simulink model "gtm_design"  (R2021b)
settings: Solver=VariableStepAuto  StartTime=0.0  StopTime=10.0  MinStep=0.00999  RelTol=1e-3
StopFcn:
  | MWSout=grabmws(bdroot);
  | MWSout.lastrun=datestr(now);
values from neighbouring files (symbols this model uses):
  knots2fps = 1.68781    [setup.m]
  s = tf('s')    [setup.m]
undefined symbols (not defined in the file or in its folder): Aero, aftfuel, aftfuel_pos, AILL, AILLC, AILR, AILRC, alpha_deg, alt0, altitude_ft, Ax_g, Ay_g, Az_g, b, beta_deg, bias, BRAKEC, Cbar, cg_pos0, cg_shift_gear, ControlMode, DamageCase, DamageModels, DamageOnsetTime, deltc, Earth, ELLIB, ELLIBC, ELLOB, ELLOBC, ELRIB, ELRIBC, ELROB, ELROBC, engl_ang, engl_pos, engr_ang, engr_pos, etas0, etas1, etasc_feedthrough, FLAPLC, FLAPLIB, FLAPLOB, FLAPRC, FLAPRIB, FLAPROB, FlightMode, FuelUsed_Init, fwdfuel, fwdfuel_pos, GEAR, GEARC, Inertia0, Inertia_shift_gear, Ixx_model, Iyy_model, Izz_model, KTAS, LandingGear ... (+66)
libraries: simulink_extras x98, LPVBlockLibrary x54, simulink_need_slupdate x30, aerolibconvert2 x27, simulink x7, aerolibtransform2 x6, uavalgslib x4, UserContent_lib x2, robotcorelib x1, uavutilslib x1
(part 5 of 9)

== system gtm_design/Guidance/Heading Control/FlightState ==
  Feedback : Inport
  Bus Creator : BusCreator  Inputs=8
  Bus Selector : BusSelector  OutputSignals=AirData.KTAS
  Bus Selector1 : BusSelector  OutputSignals=MIDG.NAV_Vu_mps,MIDG.NAV_Vn_mps,MIDG.NAV_Ve_mps
  Bus Selector2 : BusSelector  OutputSignals=MIDG.NAV_Ve_mps,MIDG.NAV_Vn_mps
  Bus Selector3 : BusSelector  OutputSignals=MIDG.NAV_latitude_deg,MIDG.NAV_longitude_deg,MIDG.NAV_altitude_m
  Bus Selector4 : BusSelector  OutputSignals=MIDG.phi_deg,MAG3.p_deg
  Bus to Vector : BusToVector
  Bus to Vector1 : BusToVector
  Bus to Vector2 : BusToVector
  Constant1 : Constant  Value=[37.827926944;-75.494061666]
  Constant2 : Constant  Value=0
  Constant3 : Constant  Value=0
  Degrees to Radians{,1..3} (4 alike) : simulink_extras/Transformations/Degrees to Radians
  Demux1 : Demux  Outputs=3
      settings: DisplayOption=none
  Gain : Gain  Gain=-1
  LLA to Flat Earth : aerolibtransform2/LLA to Flat Earth  units=English  ptype=Earth (WGS84)  F=1/298.257223563  R=20925646.3255  refPosPort=on  LL0=[0 10]  psi=0
      settings: SourceProductBaseCode=AE
  Map 0_1 : Subsystem
  Mux : Mux  Inputs=2
  Mux2 : Mux  Inputs=2
  Trigonometric Function1 : Trigonometry  Operator=atan2
  Trigonometric Function3 : Trigonometry  Operator=atan2
  VecNorm : Subsystem
  Velocity Conversion : aerolibconvert2/Velocity Conversion  IU=kts  OU=m/s
  fpstoknots2 : Gain  Gain=180/pi
  FlightState : Outport
  wires:
  Degrees to Radians3/1 -> Bus Creator/8  "RollAngleRate"
  Degrees to Radians2/1 -> Bus Creator/7  "RollAngle"
  Degrees to Radians1/1 -> Bus Creator/6  "FlightPathAngle"
  Degrees to Radians/1 -> Bus Creator/5  "HeadingAngle"
  Bus Creator/1 -> FlightState/1
  Velocity Conversion/1 -> Bus Creator/4  "AirSpeed"
  Bus to Vector2/1 -> Degrees to Radians3/1  "RollAngleRate"
  Bus to Vector1/1 -> Degrees to Radians2/1  "RollAngle"
  Bus to Vector/1 -> Velocity Conversion/1  "KTAS"
  Bus Selector4/1 -> Bus to Vector1/1  "<phi_deg>"
  Bus Selector4/2 -> Bus to Vector2/1  "<p_deg>"
  fpstoknots2/1 -> Degrees to Radians1/1  "FlightPathAngle"
  Bus Selector/1 -> Bus to Vector/1  "<KTAS>"
  Demux1/1 -> Bus Creator/1  "North"
  Demux1/2 -> Bus Creator/2  "East"
  Gain/1 -> Bus Creator/3  "Height"
  Bus Selector1/1 -> Trigonometric Function1/1  "<NAV_Vu_mps>"
  Bus Selector1/2 -> Mux/1  "<NAV_Vn_mps>"
  Bus Selector1/3 -> Mux/2  "<NAV_Ve_mps>"
  Trigonometric Function1/1 -> fpstoknots2/1  "gamma"
  VecNorm/1(O) -> Trigonometric Function1/2
  Mux/1 -> VecNorm/1(I)
  Constant2/1 -> LLA to Flat Earth/5
  Demux1/3 -> Gain/1  "Down"
  Bus Selector3/3 -> LLA to Flat Earth/2  "<NAV_altitude_m>"
  Constant3/1 -> LLA to Flat Earth/3
  Bus Selector3/1 -> Mux2/1  "<NAV_latitude_deg>"
  Bus Selector3/2 -> Mux2/2  "<NAV_longitude_deg>"
  Constant1/1 -> LLA to Flat Earth/4
  LLA to Flat Earth/1 -> Demux1/1
  Mux2/1 -> LLA to Flat Earth/1
  Feedback/1 -> Bus Selector3/1, Bus Selector2/1, Bus Selector1/1, Bus Selector4/1, Bus Selector/1
  Bus Selector2/1 -> Trigonometric Function3/1  "<NAV_Ve_mps>"
  Map 0_1/1(O) -> Degrees to Radians/1  "HeadingAngle"
  Trigonometric Function3/1 -> Map 0_1/1(I)  "gndtrack"
  Bus Selector2/2 -> Trigonometric Function3/2  "<NAV_Vn_mps>"

== system gtm_design/Guidance/Heading Control/Windless ==
  Bus Creator : BusCreator  Inputs=4  OutDataTypeStr=Bus: FixedWingEnvironmentBus  NonVirtualBus=on
  Constant : Constant  Value=9.8066
  Constant1 : Constant  Value=0
  Constant2 : Constant  Value=0
  Constant3 : Constant  Value=0
  Environment : Outport  VectorParamsAs1DForOutWhenUnconnected=off
  wires:
  Constant/1 -> Bus Creator/4  "Gravity"
  Bus Creator/1 -> Environment/1
  Constant1/1 -> Bus Creator/1  "WindNorth"
  Constant3/1 -> Bus Creator/3  "WindDown"
  Constant2/1 -> Bus Creator/2  "WindEast"

== system gtm_design/Guidance/Orbit Following/Subsystem1 ==
  Feedback : Inport
  Bus Creator : BusCreator  Inputs=8
  Bus Selector : BusSelector  OutputSignals=AirData.KTAS
  Bus Selector1 : BusSelector  OutputSignals=MIDG.NAV_Vu_mps,MIDG.NAV_Vn_mps,MIDG.NAV_Ve_mps
  Bus Selector2 : BusSelector  OutputSignals=MIDG.NAV_Ve_mps,MIDG.NAV_Vn_mps
  Bus Selector3 : BusSelector  OutputSignals=MIDG.NAV_latitude_deg,MIDG.NAV_longitude_deg,MIDG.NAV_altitude_m
  Bus Selector4 : BusSelector  OutputSignals=MIDG.phi_deg,MAG3.p_deg
  Bus Selector6 : BusSelector  OutputSignals=North,East,Height,HeadingAngle  OutputAsBus=on
  Bus to Vector : BusToVector
  Bus to Vector1 : BusToVector
  Bus to Vector2 : BusToVector
  Constant1 : Constant  Value=[37.827926944;-75.494061666]
  Constant2 : Constant  Value=0
  Constant3 : Constant  Value=0
  Degrees to Radians{,1..3} (4 alike) : simulink_extras/Transformations/Degrees to Radians
  Demux1 : Demux  Outputs=3
      settings: DisplayOption=none
  Gain : Gain  Gain=-1
  LLA to Flat Earth : aerolibtransform2/LLA to Flat Earth  units=English  ptype=Earth (WGS84)  F=1/298.257223563  R=20925646.3255  refPosPort=on  LL0=[0 10]  psi=0
      settings: SourceProductBaseCode=AE
  Map 0_1 : Subsystem
  Mux : Mux  Inputs=2
  Mux2 : Mux  Inputs=2
  Trigonometric Function1 : Trigonometry  Operator=atan2
  Trigonometric Function3 : Trigonometry  Operator=atan2
  VecNorm : Subsystem
  Velocity Conversion : aerolibconvert2/Velocity Conversion  IU=kts  OU=m/s
  fpstoknots2 : Gain  Gain=180/pi
  Out2 : Outport
  Out1 : Outport  Port=2
  wires:
  Bus Selector2/2 -> Trigonometric Function3/2  "<NAV_Vn_mps>"
  Trigonometric Function3/1 -> Map 0_1/1(I)  "gndtrack"
  Map 0_1/1(O) -> Degrees to Radians/1  "HeadingAngle"
  Bus Selector2/1 -> Trigonometric Function3/1  "<NAV_Ve_mps>"
  Feedback/1 -> Bus Selector/1, Bus Selector4/1, Bus Selector1/1, Bus Selector2/1, Bus Selector3/1
  Mux2/1 -> LLA to Flat Earth/1
  LLA to Flat Earth/1 -> Demux1/1
  Constant1/1 -> LLA to Flat Earth/4
  Bus Selector3/2 -> Mux2/2  "<NAV_longitude_deg>"
  Bus Selector3/1 -> Mux2/1  "<NAV_latitude_deg>"
  Constant3/1 -> LLA to Flat Earth/3
  Bus Selector3/3 -> LLA to Flat Earth/2  "<NAV_altitude_m>"
  Demux1/3 -> Gain/1  "Down"
  Constant2/1 -> LLA to Flat Earth/5
  Mux/1 -> VecNorm/1(I)
  VecNorm/1(O) -> Trigonometric Function1/2
  Trigonometric Function1/1 -> fpstoknots2/1  "gamma"
  Bus Selector1/3 -> Mux/2  "<NAV_Ve_mps>"
  Bus Selector1/2 -> Mux/1  "<NAV_Vn_mps>"
  Bus Selector1/1 -> Trigonometric Function1/1  "<NAV_Vu_mps>"
  Gain/1 -> Bus Creator/3  "Height"
  Demux1/2 -> Bus Creator/2  "East"
  Demux1/1 -> Bus Creator/1  "North"
  Bus Selector/1 -> Bus to Vector/1  "<KTAS>"
  fpstoknots2/1 -> Degrees to Radians1/1  "FlightPathAngle"
  Bus Selector4/2 -> Bus to Vector2/1  "<p_deg>"
  Bus Selector4/1 -> Bus to Vector1/1  "<phi_deg>"
  Bus to Vector/1 -> Velocity Conversion/1  "KTAS"
  Bus to Vector1/1 -> Degrees to Radians2/1  "RollAngle"
  Bus to Vector2/1 -> Degrees to Radians3/1  "RollAngleRate"
  Velocity Conversion/1 -> Bus Creator/4  "AirSpeed"
  Bus Selector6/1 -> Out1/1
  Bus Creator/1 -> Bus Selector6/1, Out2/1
  Degrees to Radians/1 -> Bus Creator/5  "HeadingAngle"
  Degrees to Radians1/1 -> Bus Creator/6  "FlightPathAngle"
  Degrees to Radians2/1 -> Bus Creator/7  "RollAngle"
  Degrees to Radians3/1 -> Bus Creator/8  "RollAngleRate"

== system gtm_design/Guidance/Orbit Following/Windless ==
  Bus Creator : BusCreator  Inputs=4  OutDataTypeStr=Bus: FixedWingEnvironmentBus  NonVirtualBus=on
  Constant : Constant  Value=9.8066
  Constant1 : Constant  Value=0
  Constant2 : Constant  Value=0
  Constant3 : Constant  Value=0
  Environment : Outport  VectorParamsAs1DForOutWhenUnconnected=off
  wires:
  Constant2/1 -> Bus Creator/2  "WindEast"
  Constant3/1 -> Bus Creator/3  "WindDown"
  Constant1/1 -> Bus Creator/1  "WindNorth"
  Bus Creator/1 -> Environment/1
  Constant/1 -> Bus Creator/4  "Gravity"

== system gtm_design/Guidance/Waypoint Following/Subsystem1 ==
  Feedback : Inport
  Bus Creator : BusCreator  Inputs=8
  Bus Selector : BusSelector  OutputSignals=AirData.KTAS
  Bus Selector1 : BusSelector  OutputSignals=MIDG.NAV_Vu_mps,MIDG.NAV_Vn_mps,MIDG.NAV_Ve_mps
  Bus Selector2 : BusSelector  OutputSignals=MIDG.NAV_Ve_mps,MIDG.NAV_Vn_mps
  Bus Selector3 : BusSelector  OutputSignals=MIDG.NAV_latitude_deg,MIDG.NAV_longitude_deg,MIDG.NAV_altitude_m
  Bus Selector4 : BusSelector  OutputSignals=MIDG.phi_deg,MAG3.p_deg
  Bus Selector6 : BusSelector  OutputSignals=North,East,Height,HeadingAngle  OutputAsBus=on
  Bus to Vector : BusToVector
  Bus to Vector1 : BusToVector
  Bus to Vector2 : BusToVector
  Constant1 : Constant  Value=[37.827926944;-75.494061666]
  Constant2 : Constant  Value=0
  Constant3 : Constant  Value=0
  Degrees to Radians{,1..3} (4 alike) : simulink_extras/Transformations/Degrees to Radians
  Demux1 : Demux  Outputs=3
      settings: DisplayOption=none
  Gain : Gain  Gain=-1
  LLA to Flat Earth : aerolibtransform2/LLA to Flat Earth  units=English  ptype=Earth (WGS84)  F=1/298.257223563  R=20925646.3255  refPosPort=on  LL0=[0 10]  psi=0
      settings: SourceProductBaseCode=AE
  Map 0_1 : Subsystem
  Mux : Mux  Inputs=2
  Mux2 : Mux  Inputs=2
  Trigonometric Function1 : Trigonometry  Operator=atan2
  Trigonometric Function3 : Trigonometry  Operator=atan2
  VecNorm : Subsystem
  Velocity Conversion : aerolibconvert2/Velocity Conversion  IU=kts  OU=m/s
  fpstoknots2 : Gain  Gain=180/pi
  Out2 : Outport
  Out1 : Outport  Port=2
  wires:
  Degrees to Radians3/1 -> Bus Creator/8  "RollAngleRate"
  Degrees to Radians2/1 -> Bus Creator/7  "RollAngle"
  Degrees to Radians1/1 -> Bus Creator/6  "FlightPathAngle"
  Degrees to Radians/1 -> Bus Creator/5  "HeadingAngle"
  Bus Creator/1 -> Out2/1, Bus Selector6/1
  Bus Selector6/1 -> Out1/1
  Velocity Conversion/1 -> Bus Creator/4  "AirSpeed"
  Bus to Vector2/1 -> Degrees to Radians3/1  "RollAngleRate"
  Bus to Vector1/1 -> Degrees to Radians2/1  "RollAngle"
  Bus to Vector/1 -> Velocity Conversion/1  "KTAS"
  Bus Selector4/1 -> Bus to Vector1/1  "<phi_deg>"
  Bus Selector4/2 -> Bus to Vector2/1  "<p_deg>"
  fpstoknots2/1 -> Degrees to Radians1/1  "FlightPathAngle"
  Bus Selector/1 -> Bus to Vector/1  "<KTAS>"
  Demux1/1 -> Bus Creator/1  "North"
  Demux1/2 -> Bus Creator/2  "East"
  Gain/1 -> Bus Creator/3  "Height"
  Bus Selector1/1 -> Trigonometric Function1/1  "<NAV_Vu_mps>"
  Bus Selector1/2 -> Mux/1  "<NAV_Vn_mps>"
  Bus Selector1/3 -> Mux/2  "<NAV_Ve_mps>"
  Trigonometric Function1/1 -> fpstoknots2/1  "gamma"
  VecNorm/1(O) -> Trigonometric Function1/2
  Mux/1 -> VecNorm/1(I)
  Constant2/1 -> LLA to Flat Earth/5
  Demux1/3 -> Gain/1  "Down"
  Bus Selector3/3 -> LLA to Flat Earth/2  "<NAV_altitude_m>"
  Constant3/1 -> LLA to Flat Earth/3
  Bus Selector3/1 -> Mux2/1  "<NAV_latitude_deg>"
  Bus Selector3/2 -> Mux2/2  "<NAV_longitude_deg>"
  Constant1/1 -> LLA to Flat Earth/4
  LLA to Flat Earth/1 -> Demux1/1
  Mux2/1 -> LLA to Flat Earth/1
  Feedback/1 -> Bus Selector3/1, Bus Selector2/1, Bus Selector1/1, Bus Selector4/1, Bus Selector/1
  Bus Selector2/1 -> Trigonometric Function3/1  "<NAV_Ve_mps>"
  Map 0_1/1(O) -> Degrees to Radians/1  "HeadingAngle"
  Trigonometric Function3/1 -> Map 0_1/1(I)  "gndtrack"
  Bus Selector2/2 -> Trigonometric Function3/2  "<NAV_Vn_mps>"

== system gtm_design/Guidance/Waypoint Following/Windless ==
  Bus Creator : BusCreator  Inputs=4  OutDataTypeStr=Bus: FixedWingEnvironmentBus  NonVirtualBus=on
  Constant : Constant  Value=9.8066
  Constant1 : Constant  Value=0
  Constant2 : Constant  Value=0
  Constant3 : Constant  Value=0
  Environment : Outport  VectorParamsAs1DForOutWhenUnconnected=off
  wires:
  Constant/1 -> Bus Creator/4  "Gravity"
  Bus Creator/1 -> Environment/1
  Constant1/1 -> Bus Creator/1  "WindNorth"
  Constant3/1 -> Bus Creator/3  "WindDown"
  Constant2/1 -> Bus Creator/2  "WindEast"

== system gtm_design/Control/Controller/Control Algorithm/Hinf Autopilot ==
  cmd : Inport
  feedback : Inport  Port=2
  Action Port : ActionPort  ActionPortLabel=case [ 3 ]:
  Bus Selector : BusSelector  OutputSignals=tas_c_knot,alt_c_ft,bet_c_deg,phi_c_deg  OutputAsBus=on
  Lateral-Directional Controller : Subsystem
  Longitudinal Controller : Subsystem
  Mux : Mux  Inputs=5
  CONTROLC : Outport  PortDimensions=[5 1]  InitialOutput=zeros(5,1)
  wires:
  Mux/1 -> CONTROLC/1
  Lateral-Directional Controller/1(AILC) -> Mux/3
  Lateral-Directional Controller/2(RUDC) -> Mux/4
  Longitudinal Controller/1(THROTC) -> Mux/1
  Longitudinal Controller/2(ELLC) -> Mux/2
  Lateral-Directional Controller/3(SPANAC) -> Mux/5
  feedback/1 -> Lateral-Directional Controller/2(feedback), Longitudinal Controller/2(feedback)
  Bus Selector/1 -> Lateral-Directional Controller/1(cmd_autopilot_lat), Longitudinal Controller/1(cmd_autopilot_lon)
  cmd/1 -> Bus Selector/1

== system gtm_design/Control/Controller/Control Algorithm/Hinf CAS ==
  cmd : Inport
  feedback : Inport  Port=2
  Action Port : ActionPort  ActionPortLabel=case [ 1 ]:
  Bus Selector : BusSelector  OutputSignals=an_c_g,bet_c_deg,p_c_deg  OutputAsBus=on
  Lateral-Directional Controller : Subsystem
  Longitudinal Controller : Subsystem
  Mux : Mux  Inputs=5
  CONTROLC : Outport  PortDimensions=[5 1]  InitialOutput=zeros(5,1)
  wires:
  cmd/1 -> Bus Selector/1
  Bus Selector/1 -> Longitudinal Controller/1(cmd_cas_lon), Lateral-Directional Controller/1(cmd_cas_lat)
  feedback/1 -> Longitudinal Controller/2(feedback), Lateral-Directional Controller/2(feedback)
  Lateral-Directional Controller/3(SPANAC) -> Mux/5
  Longitudinal Controller/2(ELLC) -> Mux/2
  Longitudinal Controller/1(THROTC) -> Mux/1
  Lateral-Directional Controller/2(RUDC) -> Mux/4
  Lateral-Directional Controller/1(AILC) -> Mux/3
  Mux/1 -> CONTROLC/1

== system gtm_design/Control/Controller/Control Algorithm/LPV Autopilot ==
  cmd : Inport
  feedback : Inport  Port=2
  Action Port : ActionPort  ActionPortLabel=case [ 4 ]:
  Bus Selector : BusSelector  OutputSignals=tas_c_knot,alt_c_ft,bet_c_deg,phi_c_deg  OutputAsBus=on
  Lateral-Directional Controller : Subsystem
  Longitudinal Controller : Subsystem
  Mux : Mux  Inputs=5
  CONTROLC : Outport  PortDimensions=[5 1]  InitialOutput=zeros(5,1)
  wires:
  Bus Selector/1 -> Longitudinal Controller/1(cmd_autopilot_lon), Lateral-Directional Controller/1(cmd_autopilot_lat)
  feedback/1 -> Longitudinal Controller/2(feedback), Lateral-Directional Controller/2(feedback)
  Lateral-Directional Controller/3(SPANAC) -> Mux/5
  Longitudinal Controller/2(ELLC) -> Mux/2
  Longitudinal Controller/1(THROTC) -> Mux/1
  Lateral-Directional Controller/2(RUDC) -> Mux/4
  Lateral-Directional Controller/1(AILC) -> Mux/3
  Mux/1 -> CONTROLC/1
  cmd/1 -> Bus Selector/1

== system gtm_design/Control/Controller/Control Algorithm/LPV CAS ==
  cmd : Inport
  feedback : Inport  Port=2
  Action Port : ActionPort  ActionPortLabel=case [ 2 ]:
  Bus Selector : BusSelector  OutputSignals=an_c_g,bet_c_deg,p_c_deg  OutputAsBus=on
  Lateral-Directional Controller : Subsystem
  Longitudinal Controller : Subsystem
  Mux : Mux  Inputs=5
  CONTROLC : Outport  PortDimensions=[5 1]  InitialOutput=zeros(5,1)
  wires:
  Mux/1 -> CONTROLC/1
  Lateral-Directional Controller/1(AILC) -> Mux/3
  Lateral-Directional Controller/2(RUDC) -> Mux/4
  Longitudinal Controller/1(THROTC) -> Mux/1
  Longitudinal Controller/2(ELLC) -> Mux/2
  Lateral-Directional Controller/3(SPANAC) -> Mux/5
  feedback/1 -> Lateral-Directional Controller/2(feedback), Longitudinal Controller/2(feedback)
  Bus Selector/1 -> Lateral-Directional Controller/1(cmd_cas_lat), Longitudinal Controller/1(cmd_cas_lon)
  cmd/1 -> Bus Selector/1

== system gtm_design/Control/Controller/Control Algorithm/No Control ==
  Action Port : ActionPort  ActionPortLabel=default:
  Elevator : Constant  Value=bias.elevator
  Flaps1 : Constant  Value=bias.rudder
  Flaps2 : Constant  Value=bias.aileron
  Flaps3 : Constant  Value=0
  Mux : Mux  Inputs=5
  Throttle : Constant  Value=bias.throttle
  CONTROLC : Outport  PortDimensions=[5 1]  InitialOutput=zeros(5,1)
  wires:
  Throttle/1 -> Mux/1
  Elevator/1 -> Mux/2
  Flaps2/1 -> Mux/3
  Flaps1/1 -> Mux/4
  Flaps3/1 -> Mux/5
  Mux/1 -> CONTROLC/1

== system gtm_design/GTM_T2/A//C parameters/Inertia//Mass//CG Shift/DamageEffects ==
  In : Inport
  Gain1 : Constant  Value=dInertiaDamage
  Squeeze2 : Squeeze
  Value(ndx,:) : Selector  NumberOfDimensions=2  IndexMode=Zero-based  InputPortWidth=3  IndexOptions=Index vector (port),Select all  Indices=[1 3],1  OutputSizes=1,1
  dInertia : Outport
  wires:
  Squeeze2/1 -> dInertia/1
  Value(ndx,:)/1 -> Squeeze2/1
  Gain1/1 -> Value(ndx,:)/1
  In/1 -> Value(ndx,:)/2

== system gtm_design/GTM_T2/A//C parameters/Inertia//Mass//CG Shift/FuelBurnEffects ==
  In : Inport
  Mux : Mux
  Polyval : Subsystem  mask{p=Ixx_model}
      mask prompts: p "Polynomial"
      mask help:
      | Embedded MATLAB version of the polyval block.
      | Input polynomial coefficients as a vector in descending order.
      mask Display:
      | disp('y = P(u)\n')
      | disp(['\nO(P) = ' num2str(length(p)-1)])
  Polyval1 : Subsystem  mask{p=Iyy_model}
      mask prompts: p "Polynomial"
      mask help:
      | Embedded MATLAB version of the polyval block.
      | Input polynomial coefficients as a vector in descending order.
      mask Display:
      | disp('y = P(u)\n')
      | disp(['\nO(P) = ' num2str(length(p)-1)])
  Polyval2 : Subsystem  mask{p=Izz_model}
      mask prompts: p "Polynomial"
      mask help:
      | Embedded MATLAB version of the polyval block.
      | Input polynomial coefficients as a vector in descending order.
      mask Display:
      | disp('y = P(u)\n')
      | disp(['\nO(P) = ' num2str(length(p)-1)])
  xCG6 : Constant  Value=zeros(1,3)
  dInertia : Outport
  wires:
  Mux/1 -> dInertia/1
  Polyval2/1(Out1) -> Mux/3
  Polyval1/1(Out1) -> Mux/2
  Polyval/1(Out1) -> Mux/1
  xCG6/1 -> Mux/4
  In/1 -> Polyval2/1(In1), Polyval1/1(In1), Polyval/1(In1)

== system gtm_design/GTM_T2/A//C parameters/Inertia//Mass//CG Shift/MorphingEffects ==
  morphing : Inport
  MorphingEffectsInertia : MATLAB Function  TreatAsAtomicUnit=on
  dInertia : Outport
  dCG : Outport  Port=2
  wires:
  morphing/1 -> MorphingEffectsInertia/1(eta)
  MorphingEffectsInertia/1(dinertia) -> dInertia/1
  MorphingEffectsInertia/2(dCG) -> dCG/1

== system gtm_design/GTM_T2/A//C parameters/Inertia//Mass//CG Shift/cg//weight ==
  DamageCase : Inport
  Gain1 : Constant  Value=dMassDamage
  Gain2 : Constant  Value=dCGDamage
  Squeeze1 : Squeeze
  Squeeze2 : Squeeze
  Value(ndx,:) : Selector  IndexMode=Zero-based  IndexOptions=Index vector (port)  Indices=[1 3]  OutputSizes=1
  Value(ndx,:)1 : Selector  NumberOfDimensions=2  IndexMode=Zero-based  InputPortWidth=3  IndexOptions=Index vector (port),Select all  Indices=[1 3],1  OutputSizes=1,1
  dCG : Outport
  dweight : Outport  Port=2
  wires:
  Squeeze2/1 -> dweight/1
  Squeeze1/1 -> dCG/1
  Value(ndx,:)/1 -> Squeeze2/1
  Gain1/1 -> Value(ndx,:)/1
  DamageCase/1 -> Value(ndx,:)1/2, Value(ndx,:)/2
  Value(ndx,:)1/1 -> Squeeze1/1
  Gain2/1 -> Value(ndx,:)1/1

== system gtm_design/GTM_T2/Actuators/Acutator Dynamics/ElevatorLIBServo ==
  In : Inport
  Constant : Constant  Value=Bias
  Gain : Gain  Gain=2*pi*freq  SaturateOnIntegerOverflow=on  OutDataTypeStr=Inherit: Same as input  ParamDataTypeStr=Inherit: Same as input
  Integrator : Integrator  InitialConditionSource=external  LimitOutput=on  UpperSaturationLimit=POS_hi  LowerSaturationLimit=POS_lo  IgnoreLimit=on
  Rate Limiter : Saturate  UpperLimit=RL  LowerLimit=-RL
  Sum : Sum  Inputs=-+|  InputSameDT=on  SaturateOnIntegerOverflow=on  OutDataTypeStr=Inherit: Same as first input
  Sum1 : Sum  Inputs=++|  InputSameDT=on  SaturateOnIntegerOverflow=on  OutDataTypeStr=Inherit: Same as first input
  Out : Outport  PortDimensions=1
  wires:
  Constant/1 -> Sum1/1
  Sum1/1 -> Integrator/2, Sum/2
  In/1 -> Sum1/2
  Rate Limiter/1 -> Integrator/1  "Ydot_lim"
  Integrator/1 -> Out/1, Sum/1  "Y"
  Sum/1 -> Gain/1  "Error"
  Gain/1 -> Rate Limiter/1  "Ydot"

== system gtm_design/GTM_T2/Actuators/Acutator Dynamics/ElevatorLOBServo ==
  In : Inport
  Constant : Constant  Value=Bias
  Gain : Gain  Gain=2*pi*freq  SaturateOnIntegerOverflow=on  OutDataTypeStr=Inherit: Same as input  ParamDataTypeStr=Inherit: Same as input
  Integrator : Integrator  InitialConditionSource=external  LimitOutput=on  UpperSaturationLimit=POS_hi  LowerSaturationLimit=POS_lo  IgnoreLimit=on
  Rate Limiter : Saturate  UpperLimit=RL  LowerLimit=-RL
  Sum : Sum  Inputs=-+|  InputSameDT=on  SaturateOnIntegerOverflow=on  OutDataTypeStr=Inherit: Same as first input
  Sum1 : Sum  Inputs=++|  InputSameDT=on  SaturateOnIntegerOverflow=on  OutDataTypeStr=Inherit: Same as first input
  Out : Outport  PortDimensions=1
  wires:
  Constant/1 -> Sum1/1
  Sum1/1 -> Integrator/2, Sum/2
  In/1 -> Sum1/2
  Rate Limiter/1 -> Integrator/1  "Ydot_lim"
  Integrator/1 -> Out/1, Sum/1  "Y"
  Sum/1 -> Gain/1  "Error"
  Gain/1 -> Rate Limiter/1  "Ydot"

== system gtm_design/GTM_T2/Actuators/Acutator Dynamics/ElevatorRIBServo ==
  In : Inport
  Constant : Constant  Value=Bias
  Gain : Gain  Gain=2*pi*freq  SaturateOnIntegerOverflow=on  OutDataTypeStr=Inherit: Same as input  ParamDataTypeStr=Inherit: Same as input
  Integrator : Integrator  InitialConditionSource=external  LimitOutput=on  UpperSaturationLimit=POS_hi  LowerSaturationLimit=POS_lo  IgnoreLimit=on
  Rate Limiter : Saturate  UpperLimit=RL  LowerLimit=-RL
  Sum : Sum  Inputs=-+|  InputSameDT=on  SaturateOnIntegerOverflow=on  OutDataTypeStr=Inherit: Same as first input
  Sum1 : Sum  Inputs=++|  InputSameDT=on  SaturateOnIntegerOverflow=on  OutDataTypeStr=Inherit: Same as first input
  Out : Outport  PortDimensions=1
  wires:
  Constant/1 -> Sum1/1
  Sum1/1 -> Integrator/2, Sum/2
  In/1 -> Sum1/2
  Rate Limiter/1 -> Integrator/1  "Ydot_lim"
  Integrator/1 -> Out/1, Sum/1  "Y"
  Sum/1 -> Gain/1  "Error"
  Gain/1 -> Rate Limiter/1  "Ydot"

== system gtm_design/GTM_T2/Actuators/Acutator Dynamics/ElevatorROBServo ==
  In : Inport
  Constant : Constant  Value=Bias
  Gain : Gain  Gain=2*pi*freq  SaturateOnIntegerOverflow=on  OutDataTypeStr=Inherit: Same as input  ParamDataTypeStr=Inherit: Same as input
  Integrator : Integrator  InitialConditionSource=external  LimitOutput=on  UpperSaturationLimit=POS_hi  LowerSaturationLimit=POS_lo  IgnoreLimit=on
  Rate Limiter : Saturate  UpperLimit=RL  LowerLimit=-RL
  Sum : Sum  Inputs=-+|  InputSameDT=on  SaturateOnIntegerOverflow=on  OutDataTypeStr=Inherit: Same as first input
  Sum1 : Sum  Inputs=++|  InputSameDT=on  SaturateOnIntegerOverflow=on  OutDataTypeStr=Inherit: Same as first input
  Out : Outport  PortDimensions=1
  wires:
  Constant/1 -> Sum1/1
  Sum1/1 -> Integrator/2, Sum/2
  In/1 -> Sum1/2
  Rate Limiter/1 -> Integrator/1  "Ydot_lim"
  Integrator/1 -> Out/1, Sum/1  "Y"
  Sum/1 -> Gain/1  "Error"
  Gain/1 -> Rate Limiter/1  "Ydot"

== system gtm_design/GTM_T2/Actuators/Acutator Dynamics/FlapLServo ==
  In : Inport
  Constant : Constant  Value=Bias
  Gain : Gain  Gain=2*pi*freq  SaturateOnIntegerOverflow=on  OutDataTypeStr=Inherit: Same as input  ParamDataTypeStr=Inherit: Same as input
  Integrator : Integrator  InitialConditionSource=external  LimitOutput=on  UpperSaturationLimit=POS_hi  LowerSaturationLimit=POS_lo  IgnoreLimit=on
  Rate Limiter : Saturate  UpperLimit=RL  LowerLimit=-RL
  Sum : Sum  Inputs=-+|  InputSameDT=on  SaturateOnIntegerOverflow=on  OutDataTypeStr=Inherit: Same as first input
  Sum1 : Sum  Inputs=++|  InputSameDT=on  SaturateOnIntegerOverflow=on  OutDataTypeStr=Inherit: Same as first input
  Out : Outport  PortDimensions=1
  wires:
  Constant/1 -> Sum1/1
  Sum1/1 -> Integrator/2, Sum/2
  In/1 -> Sum1/2
  Rate Limiter/1 -> Integrator/1  "Ydot_lim"
  Integrator/1 -> Out/1, Sum/1  "Y"
  Sum/1 -> Gain/1  "Error"
  Gain/1 -> Rate Limiter/1  "Ydot"

== system gtm_design/GTM_T2/Actuators/Acutator Dynamics/FlapRServo ==
  In : Inport
  Constant : Constant  Value=Bias
  Gain : Gain  Gain=2*pi*freq  SaturateOnIntegerOverflow=on  OutDataTypeStr=Inherit: Same as input  ParamDataTypeStr=Inherit: Same as input
  Integrator : Integrator  InitialConditionSource=external  LimitOutput=on  UpperSaturationLimit=POS_hi  LowerSaturationLimit=POS_lo  IgnoreLimit=on
  Rate Limiter : Saturate  UpperLimit=RL  LowerLimit=-RL
  Sum : Sum  Inputs=-+|  InputSameDT=on  SaturateOnIntegerOverflow=on  OutDataTypeStr=Inherit: Same as first input
  Sum1 : Sum  Inputs=++|  InputSameDT=on  SaturateOnIntegerOverflow=on  OutDataTypeStr=Inherit: Same as first input
  Out : Outport  PortDimensions=1
  wires:
  Constant/1 -> Sum1/1
  Sum1/1 -> Integrator/2, Sum/2
  In/1 -> Sum1/2
  Rate Limiter/1 -> Integrator/1  "Ydot_lim"
  Integrator/1 -> Out/1, Sum/1  "Y"
  Sum/1 -> Gain/1  "Error"
  Gain/1 -> Rate Limiter/1  "Ydot"

== system gtm_design/GTM_T2/Actuators/Acutator Dynamics/LeftAileronServo ==
  In : Inport
  Constant : Constant  Value=Bias
  Gain : Gain  Gain=2*pi*freq  SaturateOnIntegerOverflow=on  OutDataTypeStr=Inherit: Same as input  ParamDataTypeStr=Inherit: Same as input
  Integrator : Integrator  InitialConditionSource=external  LimitOutput=on  UpperSaturationLimit=POS_hi  LowerSaturationLimit=POS_lo  IgnoreLimit=on
  Rate Limiter : Saturate  UpperLimit=RL  LowerLimit=-RL
  Sum : Sum  Inputs=-+|  InputSameDT=on  SaturateOnIntegerOverflow=on  OutDataTypeStr=Inherit: Same as first input
  Sum1 : Sum  Inputs=++|  InputSameDT=on  SaturateOnIntegerOverflow=on  OutDataTypeStr=Inherit: Same as first input
  Out : Outport  PortDimensions=1
  wires:
  Constant/1 -> Sum1/1
  Sum1/1 -> Integrator/2, Sum/2
  In/1 -> Sum1/2
  Rate Limiter/1 -> Integrator/1  "Ydot_lim"
  Integrator/1 -> Out/1, Sum/1  "Y"
  Sum/1 -> Gain/1  "Error"
  Gain/1 -> Rate Limiter/1  "Ydot"

== system gtm_design/GTM_T2/Actuators/Acutator Dynamics/LeftIBSpoilerServo ==
  In : Inport
  Constant : Constant  Value=Bias
  Gain : Gain  Gain=2*pi*freq  SaturateOnIntegerOverflow=on  OutDataTypeStr=Inherit: Same as input  ParamDataTypeStr=Inherit: Same as input
  Integrator : Integrator  InitialConditionSource=external  LimitOutput=on  UpperSaturationLimit=POS_hi  LowerSaturationLimit=POS_lo  IgnoreLimit=on
  Rate Limiter : Saturate  UpperLimit=RL  LowerLimit=-RL
  Sum : Sum  Inputs=-+|  InputSameDT=on  SaturateOnIntegerOverflow=on  OutDataTypeStr=Inherit: Same as first input
  Sum1 : Sum  Inputs=++|  InputSameDT=on  SaturateOnIntegerOverflow=on  OutDataTypeStr=Inherit: Same as first input
  Out : Outport  PortDimensions=1
  wires:
  Constant/1 -> Sum1/1
  Sum1/1 -> Integrator/2, Sum/2
  In/1 -> Sum1/2
  Rate Limiter/1 -> Integrator/1  "Ydot_lim"
  Integrator/1 -> Out/1, Sum/1  "Y"
  Sum/1 -> Gain/1  "Error"
  Gain/1 -> Rate Limiter/1  "Ydot"

== system gtm_design/GTM_T2/Actuators/Acutator Dynamics/LeftOBSpoilerServo ==
  In : Inport
  Constant : Constant  Value=Bias
  Gain : Gain  Gain=2*pi*freq  SaturateOnIntegerOverflow=on  OutDataTypeStr=Inherit: Same as input  ParamDataTypeStr=Inherit: Same as input
  Integrator : Integrator  InitialConditionSource=external  LimitOutput=on  UpperSaturationLimit=POS_hi  LowerSaturationLimit=POS_lo  IgnoreLimit=on
  Rate Limiter : Saturate  UpperLimit=RL  LowerLimit=-RL
  Sum : Sum  Inputs=-+|  InputSameDT=on  SaturateOnIntegerOverflow=on  OutDataTypeStr=Inherit: Same as first input
  Sum1 : Sum  Inputs=++|  InputSameDT=on  SaturateOnIntegerOverflow=on  OutDataTypeStr=Inherit: Same as first input
  Out : Outport  PortDimensions=1
  wires:
  Constant/1 -> Sum1/1
  Sum1/1 -> Integrator/2, Sum/2
  In/1 -> Sum1/2
  Rate Limiter/1 -> Integrator/1  "Ydot_lim"
  Integrator/1 -> Out/1, Sum/1  "Y"
  Sum/1 -> Gain/1  "Error"
  Gain/1 -> Rate Limiter/1  "Ydot"

== system gtm_design/GTM_T2/Actuators/Acutator Dynamics/LeftSpanServo ==
  In : Inport
  Constant : Constant  Value=Bias
  Gain : Gain  Gain=2*pi*freq  SaturateOnIntegerOverflow=on  OutDataTypeStr=Inherit: Same as input  ParamDataTypeStr=Inherit: Same as input
  Integrator : Integrator  InitialConditionSource=external  LimitOutput=on  UpperSaturationLimit=POS_hi  LowerSaturationLimit=POS_lo  IgnoreLimit=on
  Rate Limiter : Saturate  UpperLimit=RL  LowerLimit=-RL
  Sum : Sum  Inputs=-+|  InputSameDT=on  SaturateOnIntegerOverflow=on  OutDataTypeStr=Inherit: Same as first input
  Sum1 : Sum  Inputs=++|  InputSameDT=on  SaturateOnIntegerOverflow=on  OutDataTypeStr=Inherit: Same as first input
  Out : Outport  PortDimensions=1
  wires:
  Gain/1 -> Rate Limiter/1  "Ydot"
  Sum/1 -> Gain/1  "Error"
  Integrator/1 -> Sum/1, Out/1  "Y"
  Rate Limiter/1 -> Integrator/1  "Ydot_lim"
  In/1 -> Sum1/2
  Sum1/1 -> Sum/2, Integrator/2
  Constant/1 -> Sum1/1

== system gtm_design/GTM_T2/Actuators/Acutator Dynamics/RightAileronServo ==
  In : Inport
  Constant : Constant  Value=Bias
  Gain : Gain  Gain=2*pi*freq  SaturateOnIntegerOverflow=on  OutDataTypeStr=Inherit: Same as input  ParamDataTypeStr=Inherit: Same as input
  Integrator : Integrator  InitialConditionSource=external  LimitOutput=on  UpperSaturationLimit=POS_hi  LowerSaturationLimit=POS_lo  IgnoreLimit=on
  Rate Limiter : Saturate  UpperLimit=RL  LowerLimit=-RL
  Sum : Sum  Inputs=-+|  InputSameDT=on  SaturateOnIntegerOverflow=on  OutDataTypeStr=Inherit: Same as first input
  Sum1 : Sum  Inputs=++|  InputSameDT=on  SaturateOnIntegerOverflow=on  OutDataTypeStr=Inherit: Same as first input
  Out : Outport  PortDimensions=1
  wires:
  Constant/1 -> Sum1/1
  Sum1/1 -> Integrator/2, Sum/2
  In/1 -> Sum1/2
  Rate Limiter/1 -> Integrator/1  "Ydot_lim"
  Integrator/1 -> Out/1, Sum/1  "Y"
  Sum/1 -> Gain/1  "Error"
  Gain/1 -> Rate Limiter/1  "Ydot"

== system gtm_design/GTM_T2/Actuators/Acutator Dynamics/RightIBSpoilerServo ==
  In : Inport
  Constant : Constant  Value=Bias
  Gain : Gain  Gain=2*pi*freq  SaturateOnIntegerOverflow=on  OutDataTypeStr=Inherit: Same as input  ParamDataTypeStr=Inherit: Same as input
  Integrator : Integrator  InitialConditionSource=external  LimitOutput=on  UpperSaturationLimit=POS_hi  LowerSaturationLimit=POS_lo  IgnoreLimit=on
  Rate Limiter : Saturate  UpperLimit=RL  LowerLimit=-RL
  Sum : Sum  Inputs=-+|  InputSameDT=on  SaturateOnIntegerOverflow=on  OutDataTypeStr=Inherit: Same as first input
  Sum1 : Sum  Inputs=++|  InputSameDT=on  SaturateOnIntegerOverflow=on  OutDataTypeStr=Inherit: Same as first input
  Out : Outport  PortDimensions=1
  wires:
  Constant/1 -> Sum1/1
  Sum1/1 -> Integrator/2, Sum/2
  In/1 -> Sum1/2
  Rate Limiter/1 -> Integrator/1  "Ydot_lim"
  Integrator/1 -> Out/1, Sum/1  "Y"
  Sum/1 -> Gain/1  "Error"
  Gain/1 -> Rate Limiter/1  "Ydot"

== system gtm_design/GTM_T2/Actuators/Acutator Dynamics/RightOBSpoilerServo ==
  In : Inport
  Constant : Constant  Value=Bias
  Gain : Gain  Gain=2*pi*freq  SaturateOnIntegerOverflow=on  OutDataTypeStr=Inherit: Same as input  ParamDataTypeStr=Inherit: Same as input
  Integrator : Integrator  InitialConditionSource=external  LimitOutput=on  UpperSaturationLimit=POS_hi  LowerSaturationLimit=POS_lo  IgnoreLimit=on
  Rate Limiter : Saturate  UpperLimit=RL  LowerLimit=-RL
  Sum : Sum  Inputs=-+|  InputSameDT=on  SaturateOnIntegerOverflow=on  OutDataTypeStr=Inherit: Same as first input
  Sum1 : Sum  Inputs=++|  InputSameDT=on  SaturateOnIntegerOverflow=on  OutDataTypeStr=Inherit: Same as first input
  Out : Outport  PortDimensions=1
  wires:
  Constant/1 -> Sum1/1
  Sum1/1 -> Integrator/2, Sum/2
  In/1 -> Sum1/2
  Rate Limiter/1 -> Integrator/1  "Ydot_lim"
  Integrator/1 -> Out/1, Sum/1  "Y"
  Sum/1 -> Gain/1  "Error"
  Gain/1 -> Rate Limiter/1  "Ydot"

== system gtm_design/GTM_T2/Actuators/Acutator Dynamics/RightSpanServo ==
  In : Inport
  Constant : Constant  Value=Bias
  Gain : Gain  Gain=2*pi*freq  SaturateOnIntegerOverflow=on  OutDataTypeStr=Inherit: Same as input  ParamDataTypeStr=Inherit: Same as input
  Integrator : Integrator  InitialConditionSource=external  LimitOutput=on  UpperSaturationLimit=POS_hi  LowerSaturationLimit=POS_lo  IgnoreLimit=on
  Rate Limiter : Saturate  UpperLimit=RL  LowerLimit=-RL
  Sum : Sum  Inputs=-+|  InputSameDT=on  SaturateOnIntegerOverflow=on  OutDataTypeStr=Inherit: Same as first input
  Sum1 : Sum  Inputs=++|  InputSameDT=on  SaturateOnIntegerOverflow=on  OutDataTypeStr=Inherit: Same as first input
  Out : Outport  PortDimensions=1
  wires:
  Gain/1 -> Rate Limiter/1  "Ydot"
  Sum/1 -> Gain/1  "Error"
  Integrator/1 -> Sum/1, Out/1  "Y"
  Rate Limiter/1 -> Integrator/1  "Ydot_lim"
  In/1 -> Sum1/2
  Sum1/1 -> Sum/2, Integrator/2
  Constant/1 -> Sum1/1

== system gtm_design/GTM_T2/Actuators/Acutator Dynamics/RudderLServo ==
  In : Inport
  Constant : Constant  Value=Bias
  Gain : Gain  Gain=2*pi*freq  SaturateOnIntegerOverflow=on  OutDataTypeStr=Inherit: Same as input  ParamDataTypeStr=Inherit: Same as input
  Integrator : Integrator  InitialConditionSource=external  LimitOutput=on  UpperSaturationLimit=POS_hi  LowerSaturationLimit=POS_lo  IgnoreLimit=on
  Rate Limiter : Saturate  UpperLimit=RL  LowerLimit=-RL
  Sum : Sum  Inputs=-+|  InputSameDT=on  SaturateOnIntegerOverflow=on  OutDataTypeStr=Inherit: Same as first input
  Sum1 : Sum  Inputs=++|  InputSameDT=on  SaturateOnIntegerOverflow=on  OutDataTypeStr=Inherit: Same as first input
  Out : Outport  PortDimensions=1
  wires:
  Constant/1 -> Sum1/1
  Sum1/1 -> Integrator/2, Sum/2
  In/1 -> Sum1/2
  Rate Limiter/1 -> Integrator/1  "Ydot_lim"
  Integrator/1 -> Out/1, Sum/1  "Y"
  Sum/1 -> Gain/1  "Error"
  Gain/1 -> Rate Limiter/1  "Ydot"

== system gtm_design/GTM_T2/Actuators/Acutator Dynamics/RudderUServo ==
  In : Inport
  Constant : Constant  Value=Bias
  Gain : Gain  Gain=2*pi*freq  SaturateOnIntegerOverflow=on  OutDataTypeStr=Inherit: Same as input  ParamDataTypeStr=Inherit: Same as input
  Integrator : Integrator  InitialConditionSource=external  LimitOutput=on  UpperSaturationLimit=POS_hi  LowerSaturationLimit=POS_lo  IgnoreLimit=on
  Rate Limiter : Saturate  UpperLimit=RL  LowerLimit=-RL
  Sum : Sum  Inputs=-+|  InputSameDT=on  SaturateOnIntegerOverflow=on  OutDataTypeStr=Inherit: Same as first input
  Sum1 : Sum  Inputs=++|  InputSameDT=on  SaturateOnIntegerOverflow=on  OutDataTypeStr=Inherit: Same as first input
  Out : Outport  PortDimensions=1
  wires:
  Constant/1 -> Sum1/1
  Sum1/1 -> Integrator/2, Sum/2
  In/1 -> Sum1/2
  Rate Limiter/1 -> Integrator/1  "Ydot_lim"
  Integrator/1 -> Out/1, Sum/1  "Y"
  Sum/1 -> Gain/1  "Error"
  Gain/1 -> Rate Limiter/1  "Ydot"

== system gtm_design/GTM_T2/Actuators/Acutator Dynamics/SteeringServo ==
  In : Inport
  Constant : Constant  Value=Bias
  Gain : Gain  Gain=2*pi*freq  SaturateOnIntegerOverflow=on  OutDataTypeStr=Inherit: Same as input  ParamDataTypeStr=Inherit: Same as input
  Integrator : Integrator  InitialConditionSource=external  LimitOutput=on  UpperSaturationLimit=POS_hi  LowerSaturationLimit=POS_lo  IgnoreLimit=on
  Rate Limiter : Saturate  UpperLimit=RL  LowerLimit=-RL
  Sum : Sum  Inputs=-+|  InputSameDT=on  SaturateOnIntegerOverflow=on  OutDataTypeStr=Inherit: Same as first input
  Sum1 : Sum  Inputs=++|  InputSameDT=on  SaturateOnIntegerOverflow=on  OutDataTypeStr=Inherit: Same as first input
  Out : Outport  PortDimensions=1
  wires:
  Constant/1 -> Sum1/1
  Sum1/1 -> Integrator/2, Sum/2
  In/1 -> Sum1/2
  Rate Limiter/1 -> Integrator/1  "Ydot_lim"
  Integrator/1 -> Out/1, Sum/1  "Y"
  Sum/1 -> Gain/1  "Error"
  Gain/1 -> Rate Limiter/1  "Ydot"

== system gtm_design/GTM_T2/Actuators/DeadBand/Deadband ==
  In : Inport
  Backlash : Backlash  Commented=on
  Bus Assignment : BusAssignment  AssignedSignals=ELLOB,ELLIB,ELROB,ELRIB,AILL,AILR,RUDU,RUDL,FLAPLIB,FLAPLOB,FLAPRIB,FLAPROB
  Bus Selector : BusSelector  OutputSignals=ELLOB,ELLIB,ELROB,ELRIB,AILL,AILR,RUDU,RUDL,FLAPLIB,FLAPLOB,FLAPRIB,FLAPROB
  Coulomb & Viscous Friction : simulink/Discontinuities/Coulomb & Viscous Friction  Commented=on  offset=[1 3 2 0]  gain=1
  Dead Zone : DeadZone  LowerValue=-0.3  UpperValue=0.3  SaturateOnIntegerOverflow=on
  Dead Zone1 : DeadZone  LowerValue=-0.6  UpperValue=0.6  SaturateOnIntegerOverflow=on
  Dead Zone{6,12..15} (5 alike) : DeadZone  LowerValue=-0.4  UpperValue=0.4  SaturateOnIntegerOverflow=on
  Dead Zone2 : DeadZone  LowerValue=-0.3  UpperValue=0.3  SaturateOnIntegerOverflow=on
  Dead Zone3 : DeadZone  LowerValue=-0.6  UpperValue=0.6  SaturateOnIntegerOverflow=on
  Dead Zone4 : DeadZone  LowerValue=-0.25  UpperValue=0.25  SaturateOnIntegerOverflow=on
  Dead Zone5 : DeadZone  LowerValue=-0.25  UpperValue=0.25  SaturateOnIntegerOverflow=on
  Dead Zone7 : DeadZone  LowerValue=-0.3  UpperValue=0.3  SaturateOnIntegerOverflow=on
  Out : Outport
  wires:
  Bus Selector/1 -> Dead Zone/1  "<ELLOB>"
  Bus Selector/2 -> Dead Zone1/1  "<ELLIB>"
  Bus Selector/3 -> Dead Zone2/1  "<ELROB>"
  Bus Selector/4 -> Dead Zone3/1  "<ELRIB>"
  Bus Selector/5 -> Dead Zone4/1  "<AILL>"
  Bus Selector/6 -> Dead Zone5/1  "<AILR>"
  Bus Selector/7 -> Dead Zone6/1  "<RUDU>"
  Bus Selector/8 -> Dead Zone7/1  "<RUDL>"
  Bus Selector/9 -> Dead Zone12/1  "<FLAPLIB>"
  Bus Selector/10 -> Dead Zone13/1  "<FLAPLOB>"
  Bus Selector/11 -> Dead Zone14/1  "<FLAPRIB>"
  Bus Selector/12 -> Dead Zone15/1  "<FLAPROB>"
  Dead Zone/1 -> Bus Assignment/2
  Dead Zone1/1 -> Bus Assignment/3
  Dead Zone2/1 -> Bus Assignment/4
  Dead Zone3/1 -> Bus Assignment/5
  Dead Zone4/1 -> Bus Assignment/6
  Dead Zone5/1 -> Bus Assignment/7
  Dead Zone6/1 -> Bus Assignment/8
  Dead Zone7/1 -> Bus Assignment/9
  Dead Zone12/1 -> Bus Assignment/10
  Dead Zone13/1 -> Bus Assignment/11
  Dead Zone14/1 -> Bus Assignment/12
  Dead Zone15/1 -> Bus Assignment/13
  In/1 -> Bus Assignment/1, Bus Selector/1
  Bus Assignment/1 -> Out/1

== system gtm_design/GTM_T2/Actuators/InputModification for Trimming/Invalid, Error Out ==
  Action Port : ActionPort  ActionPortLabel=default:
  Constant1 : Constant  Value=zeros(22,1)
  Constant2 : Constant  Value=0
  InvalidMode : Assertion  AssertionFailFcn="warndlg('Invalid settings for TrimMode and LinearizeMode.  Run setup.m to reset.','Warning!')"
  Out : Outport  InitialOutput=zeros(22,1)
  wires:
  Constant1/1 -> Out/1
  Constant2/1 -> InvalidMode/1

== system gtm_design/GTM_T2/Actuators/InputModification for Trimming/LinearizeMode:DetlasOnTrimBias ==
  In1 : Inport
  Action Port : ActionPort  ActionPortLabel=case [ 2 ]:
  Surface Allocation For Linearizing : Subsystem
  Out : Outport
  wires:
  Surface Allocation For Linearizing/1(O) -> Out/1
  In1/1 -> Surface Allocation For Linearizing/1(I)

== system gtm_design/GTM_T2/Actuators/InputModification for Trimming/SimMode:PassThroughWithStab ==
  Cmd : Inport
  Action Port : ActionPort  ActionPortLabel=case [ 0 ]:
  Demux7 : Demux  Outputs=[4+2+2+4+4, 1+1+2+1]
  Gain : Gain
  Gain1 : Gain
  Mux : Mux  Inputs=3
  Set with a wrench on T2/T3 : Constant  Value=bias.stabilizer
  Out : Outport  InitialOutput=zeros(22,1)
  wires:
  Cmd/1 -> Demux7/1
  Set with a wrench on T2/T3/1 -> Mux/2
  Mux/1 -> Out/1
  Demux7/1 -> Gain1/1  "Elevator(4)Aileron(2),Rudder(2),Spoliers(4),Flaps(4)"
  Demux7/2 -> Gain/1  "Gear,Brakes,Throttle(2),Steering"
  Gain1/1 -> Mux/1
  Gain/1 -> Mux/3

== system gtm_design/GTM_T2/Actuators/InputModification for Trimming/TrimMode: DriveFromTopLevel ==
  TrimBias : Inport
  Action Port : ActionPort  ActionPortLabel=case [ 1 ]:
  Bus Assignment : BusAssignment  AssignedSignals=ELLOB,ELLIB,ELROB,ELRIB,STAB,AILL,AILR,RUDU,RUDL,THROTL,THROTR,FLAPLIB,FLAPLOB,FLAPRIB,FLAPROB,GEAR,SPLLIB,SPLLOB,SPLRIB,SPLROB
  Constant1 : Constant  Value=TrimWithStab
  Demux : Demux
  Demux1 : Demux  Outputs=5
  Demux2 : Demux  Outputs=2
  Demux3 : Demux  Outputs=2
  Demux4 : Demux  Outputs=2
  Demux6 : Demux
  Flaps1 : Constant  Value=bias.speedbrake
  Flaps2 : Constant  Value=bias.flaps
  Flaps3 : Constant  Value=bias.flaps
  Flaps4 : Constant  Value=bias.morphing
  Flaps5 : Constant  Value=bias.morphing
  Force Consistent Sample Time on Bus : Subsystem
  Gear : Constant  Value=bias.geardown
  InitializeBus : Subsystem
  Map : Gain  Gain=[-1;1]
  Map1 : Gain  Gain=[1;1]
  Map2 : Gain  Gain=[1;1]
  Map4 : Gain  Gain=[1;1;1;1]
  MapPitchSurf : Subsystem
  Out : Outport  InitialOutput=zeros(22,1)
  wires:
  Bus Assignment/1 -> Force Consistent Sample Time on Bus/1(In1)
  Force Consistent Sample Time on Bus/1(Out1) -> Out/1
  InitializeBus/1(O) -> Bus Assignment/1
  MapPitchSurf/1(Out) -> Demux1/1
  Flaps1/1 -> Map4/1
  Gear/1 -> Bus Assignment/17
  Map1/1 -> Demux3/1
  Demux4/2 -> Bus Assignment/12
  Demux4/1 -> Bus Assignment/11
  Map2/1 -> Demux4/1
  Demux3/2 -> Bus Assignment/10
  Demux3/1 -> Bus Assignment/9
  Demux2/2 -> Bus Assignment/8
  Demux2/1 -> Bus Assignment/7
  Demux1/5 -> Bus Assignment/6
  Demux1/4 -> Bus Assignment/5
  Demux1/3 -> Bus Assignment/4
  Demux1/2 -> Bus Assignment/3
  Demux1/1 -> Bus Assignment/2
  Constant1/1 -> MapPitchSurf/1(UseStab)
  Demux/4 -> Map2/1  "Throttle"
  Demux/3 -> Map1/1  "Rudder"
  Demux/2 -> Map/1  "Aileron"
  Demux/1 -> MapPitchSurf/2(In)  "PitchSurf"
  TrimBias/1 -> Demux/1
  Map/1 -> Demux2/1
  Map4/1 -> Demux6/1
  Demux6/1 -> Bus Assignment/18
  Demux6/3 -> Bus Assignment/20
  Demux6/2 -> Bus Assignment/19
  Demux6/4 -> Bus Assignment/21
  Flaps3/1 -> Bus Assignment/13
  Flaps5/1 -> Bus Assignment/14
  Flaps4/1 -> Bus Assignment/16
  Flaps2/1 -> Bus Assignment/15

== system gtm_design/GTM_T2/Aero/Basic Airframe/DamageEffects ==
  alpha : Inport
  beta : Inport  Port=2
  damage_case : Inport  Port=3
  Merge : Merge  InitialOutput=zeros(6,1)
  Switch Case : SwitchCase  CaseConditions={[1,2,3,4,5,6]}
  Switch Case Action Subsystem : Subsystem  TreatAsAtomicUnit=on
  Switch Case Action Subsystem2 : Subsystem  TreatAsAtomicUnit=on
  damage_case_DUP : InportShadow  Port=3
  dC6_dam : Outport
  wires:
  damage_case_DUP/1 -> Switch Case Action Subsystem/3(damage_case)
  Switch Case Action Subsystem/1(dC6_dam) -> Merge/1
  Switch Case/1 -> Switch Case Action Subsystem/Action
  damage_case/1 -> Switch Case/1
  Merge/1 -> dC6_dam/1
  beta/1 -> Switch Case Action Subsystem/2(beta)
  alpha/1 -> Switch Case Action Subsystem/1(alpha)
  Switch Case Action Subsystem2/1(Zeros) -> Merge/2
  Switch Case/2 -> Switch Case Action Subsystem2/Action

== system gtm_design/GTM_T2/Aero/Coefficent Evaluation/3D Vector Cross Product ==
  A : Inport
  B : Inport  Port=2
  Demux : Demux  Outputs=3
      settings: DisplayOption=none
  Demux1 : Demux  Outputs=3
      settings: DisplayOption=none
  Gain : Gain  Gain=-1  SaturateOnIntegerOverflow=on  OutDataTypeStr=Inherit: Same as input  ParamDataTypeStr=Inherit: Same as input
  Ground : Ground
  Mux : Mux  Inputs=9
  Product : Product  Multiplication=Matrix(*)  SaturateOnIntegerOverflow=on  OutDataTypeStr=Inherit: Same as first input
  Reshape : Reshape  OutputDimensionality=Customize  OutputDimensions=[3,3]
  AxB : Outport
  wires:
  A/1 -> Demux/1, Gain/1
  Product/1 -> AxB/1
  Ground/1 -> Mux/1, Mux/5, Mux/9
  Gain/1 -> Demux1/1
  Demux/3 -> Mux/2
  Demux1/2 -> Mux/3
  Demux1/3 -> Mux/4
  Demux/1 -> Mux/6
  Demux/2 -> Mux/7
  Demux1/1 -> Mux/8
  Mux/1 -> Reshape/1
  Reshape/1 -> Product/1
  B/1 -> Product/2

== system gtm_design/GTM_T2/Aero/Control Surfaces/Ailerons ==
  alpha : Inport
  beta : Inport  Port=2
  AILL : Inport  Port=3
  AILR : Inport  Port=4
  Constant1 : Constant  Value=[0:5]  OutDataTypeStr=uint32
  Constant3 : Constant  Value=[0:5]  OutDataTypeStr=uint32
  Gain2 : Gain  Gain=-1
  Interpolation Using Prelookup : Interpolation_n-D  NumberOfTableDimensions=4  Table=Aero.dC6_ail.data  NumSelectionDims=1
      settings: InputPortMap=u0,u1,u2,u3,u4,u5,u6
  Interpolation Using Prelookup1 : Interpolation_n-D  NumberOfTableDimensions=4  Table=Aero.dC6_ail.data  NumSelectionDims=1
      settings: InputPortMap=u0,u1,u2,u3,u4,u5,u6
  Negate Lateral : Gain  Gain=[1 -1 1 -1 1 -1]
  Prelookup1 : PreLookup  BreakpointsData=Aero.dC6_ail.alpha  IndexSearchMethod=Linear search  BeginIndexSearchUsingPreviousIndexResult=on  ExtrapMethod=Linear
  Prelookup2 : PreLookup  BreakpointsData=Aero.dC6_ail.beta  IndexSearchMethod=Linear search  BeginIndexSearchUsingPreviousIndexResult=on  ExtrapMethod=Linear
  Prelookup3 : PreLookup  BreakpointsData=Aero.dC6_ail.ail  IndexSearchMethod=Linear search  BeginIndexSearchUsingPreviousIndexResult=on  ExtrapMethod=Linear
  Prelookup4 : PreLookup  BreakpointsData=Aero.dC6_ail.beta  IndexSearchMethod=Linear search  BeginIndexSearchUsingPreviousIndexResult=on  ExtrapMethod=Linear
  Prelookup5 : PreLookup  BreakpointsData=Aero.dC6_ail.ail  IndexSearchMethod=Linear search  BeginIndexSearchUsingPreviousIndexResult=on  ExtrapMethod=Linear
  Left : Outport
  Right : Outport  Port=2
  wires:
  Interpolation Using Prelookup/1 -> Negate Lateral/1
  Constant1/1 -> Interpolation Using Prelookup1/7
  Prelookup5/2 -> Interpolation Using Prelookup1/6
  Prelookup5/1 -> Interpolation Using Prelookup1/5
  Prelookup4/2 -> Interpolation Using Prelookup1/4
  Prelookup4/1 -> Interpolation Using Prelookup1/3
  Constant3/1 -> Interpolation Using Prelookup/7
  Prelookup3/2 -> Interpolation Using Prelookup/6
  Prelookup3/1 -> Interpolation Using Prelookup/5
  Prelookup2/2 -> Interpolation Using Prelookup/4
  Prelookup2/1 -> Interpolation Using Prelookup/3
  Prelookup1/2 -> Interpolation Using Prelookup1/2, Interpolation Using Prelookup/2
  Prelookup1/1 -> Interpolation Using Prelookup1/1, Interpolation Using Prelookup/1
  AILL/1 -> Prelookup3/1
  beta/1 -> Prelookup4/1, Gain2/1
  AILR/1 -> Prelookup5/1
  Gain2/1 -> Prelookup2/1
  alpha/1 -> Prelookup1/1
  Negate Lateral/1 -> Left/1
  Interpolation Using Prelookup1/1 -> Right/1
